simulink model "Lez_6_BasePerTracing"  (R2024b)
settings: Solver=FixedStepDiscrete  StartTime=0.0  StopTime=Inf  RelTol=1e-3  EnableMultiTasking=on
InitFcn:
  | mcb_pmsm_foc_qep_f28379d_data;
values from neighbouring files (symbols this model uses):
  ADCCount = ADCResolution-1    (= 4095)    [Lez_6_Parameters.m]
  dataType = 'single'    [mcb_pmsm_foc_qep_f28379d_data.m]
  GainVsense = 4.99/(62+4.99)    (= 0.0744887296611)    [Lez_6_Parameters.m]
  Km = 0.11    [Lez_6_Parameters.m]
  Kpi = L/ti    (= 41)    [Lez_6_Parameters.m]
  Kpw = J/(tm*Km)    (= 0.00376470588235)    [Lez_6_Parameters.m]
  OffsetADCINC4 = 2279    [Lez_6_Parameters.m]
  PulseNumber = 2048*4    (= 8192)    [Lez_6_Parameters.m]
  RadiantsPerCount = 2*pi/(PulseNumber-1)    (= 0.00076708403213)    [Lez_6_Parameters.m]
  RpmToRads = 2*pi/60    (= 0.10471975512)    [Lez_6_Parameters.m]
  TaoFilterOffsetCurrent = 1    [Lez_6_Parameters.m]
  TaoFilterOmega = 0.002    [Lez_6_Parameters.m]
  Tii = L/R    (= 0.00128125)    [Lez_6_Parameters.m]
  Tiw = tm    (= 0.085)    [Lez_6_Parameters.m]
  TSample = 0.0001    [Lez_6_Parameters.m]
  VrefADC = 3    [Lez_6_Parameters.m]
undefined symbols (not defined in the file or in its folder): Down, GPTRIP1SEL, GPTRIP2SEL, TZ1, TZ2, Up
libraries: c2802xlib x9, c280xlib x4, simulink x4, c2837xDlib x3, c2000lib x1, svdutilitieslib x1
(part 2 of 2)

== matlab function Lez_6_BasePerTracing/Current Control/PI Current2 ==
  data: in input; Kp input; Ti input; Ts input; out output; Enable input; HiSat input; LowSat input; EnableCheckSat input

% function out = PI( in ,Kp , Ti , Ts , Enable, HiSat, LowSat, EnableCheckSat)
% persistent in_prev out_prev 
% % Initial Value
%     if isempty( out_prev )
%     out_prev = 0;
%     end
%     if isempty( in_prev )
%     in_prev = 0;
%     end
% % G(s)=(Kp/Ti)*((1+Ti*s)/s) (Tustin)
% % We run control only if motor is running
%     if (Enable == 1)
%     %I Calculate the output
%      out = Kp*Ts/(2*Ti)*(in+in_prev) + Kp*(in-in_prev) + out_prev;
%      if(EnableCheckSat == 1)
%         %check for saturation
%         if out > HiSat
%                 out = HiSat;
%             elseif (out < LowSat)
%                 out = LowSat; 
%         end
%         %% anti windup
%         if(out>HiSat)
%             out=HiSat;
%             in =((out-out_prev)-(Kp*Ts/2/Ti/Kp)*in_prev)/(Kp*Ts/2/Ti/Kp);
%         elseif (out<LowSat)
%             out=LowSat;
%             in =((out-out_prev)-(Kp*Ts/2/Ti/Kp)*in_prev)/(Kp*Ts/2/Ti/Kp);
%         end
% 
%      end
%     else
%     out = 0;
%     in = 0;
%     end
% 
% out_prev = out;
% in_prev = in;
% 
% %saturazione provvisoria
% % % out =0;
% end

function out = PI(in, Kp, Ti, Ts, Enable, HiSat, LowSat, EnableCheckSat)
persistent in_prev out_prev

% Initial Value
if isempty(out_prev)
    out_prev = 0;
end
if isempty(in_prev)
    in_prev = 0;
end

% G(s)=(Kp/Ti)*(((1+Ti*s)/s) (Tustin)
% Eseguiamo il controllo solo se abilitato
if (Enable == 1)
    % 1. Calcolo dell'uscita (Forma incrementale del PI)
    out = (Kp*Ts/(2*Ti))*(in + in_prev) + Kp*(in - in_prev) + out_prev;
    
    % 2. Saturazione e Anti-windup integrato
    if (EnableCheckSat == 1)
        if out > HiSat
            out = HiSat;
        elseif out < LowSat
            out = LowSat;
        end
        % NOTA: L'anti-windup avviene automaticamente perché stiamo per 
        % salvare la 'out' (eventualmente saturata) dentro 'out_prev'.
    end
    
    % 3. Aggiornamento stati
    out_prev = out;
    in_prev = in;
    
else
    % Se non abilitato, uscita a zero e reset degli stati del PI
    out = 0;
    out_prev = 0;
    in_prev = 0;
end

end

== matlab function Lez_6_BasePerTracing/Current Control/PI Current3 ==
  data: in input; Kp input; Ti input; Ts input; out output; Enable input; HiSat input; LowSat input; EnableCheckSat input

% function out = PI( in ,Kp , Ti , Ts , Enable, HiSat, LowSat, EnableCheckSat)
% persistent in_prev out_prev 
% % Initial Value
%     if isempty( out_prev )
%     out_prev = 0;
%     end
%     if isempty( in_prev )
%     in_prev = 0;
%     end
% % G(s)=(Kp/Ti)*((1+Ti*s)/s) (Tustin)
% % We run control only if motor is running
%     if (Enable == 1)
%     %I Calculate the output
%      out = Kp*Ts/(2*Ti)*(in+in_prev) + Kp*(in-in_prev) + out_prev;
%      if(EnableCheckSat == 1)
%         %% check for saturation
%         if out > HiSat
%                 out = HiSat;
%             elseif (out < LowSat)
%                 out = LowSat; 
%         end
%         %% anti windup
%         if(out>HiSat)
%             out=HiSat;
%             in =((out-out_prev)-(Kp*Ts/2/Ti/Kp)*in_prev)/(Kp*Ts/2/Ti/Kp);
%         elseif (out<LowSat)
%             out=LowSat;
%             in =((out-out_prev)-(Kp*Ts/2/Ti/Kp)*in_prev)/(Kp*Ts/2/Ti/Kp);
%         end
% 
%      end
%     else
%     out = 0;
%     in = 0;
%     end
% out_prev = out;
% in_prev = in;
% 
% %saturazione provvisoria
% % % out =0;
% end


function out = PI(in, Kp, Ti, Ts, Enable, HiSat, LowSat, EnableCheckSat)
persistent in_prev out_prev

% Initial Value
if isempty(out_prev)
    out_prev = 0;
end
if isempty(in_prev)
    in_prev = 0;
end

% G(s)=(Kp/Ti)*(((1+Ti*s)/s) (Tustin)
% Eseguiamo il controllo solo se abilitato
if (Enable == 1)
    % 1. Calcolo dell'uscita (Forma incrementale del PI)
    out = (Kp*Ts/(2*Ti))*(in + in_prev) + Kp*(in - in_prev) + out_prev;
    
    % 2. Saturazione e Anti-windup integrato
    if (EnableCheckSat == 1)
        if out > HiSat
            out = HiSat;
        elseif out < LowSat
            out = LowSat;
        end
        % NOTA: L'anti-windup avviene automaticamente perché stiamo per 
        % salvare la 'out' (eventualmente saturata) dentro 'out_prev'.
    end
    
    % 3. Aggiornamento stati
    out_prev = out;
    in_prev = in;
    
else
    % Se non abilitato, uscita a zero e reset degli stati del PI
    out = 0;
    out_prev = 0;
    in_prev = 0;
end

end
